simulink model "intercept_system"  (R2026b)
settings: Solver=ode4  StopTime=50  FixedStep=0.001
libraries: simulink x1
settings Model: Creator=rohan  LastModifiedBy=rohan

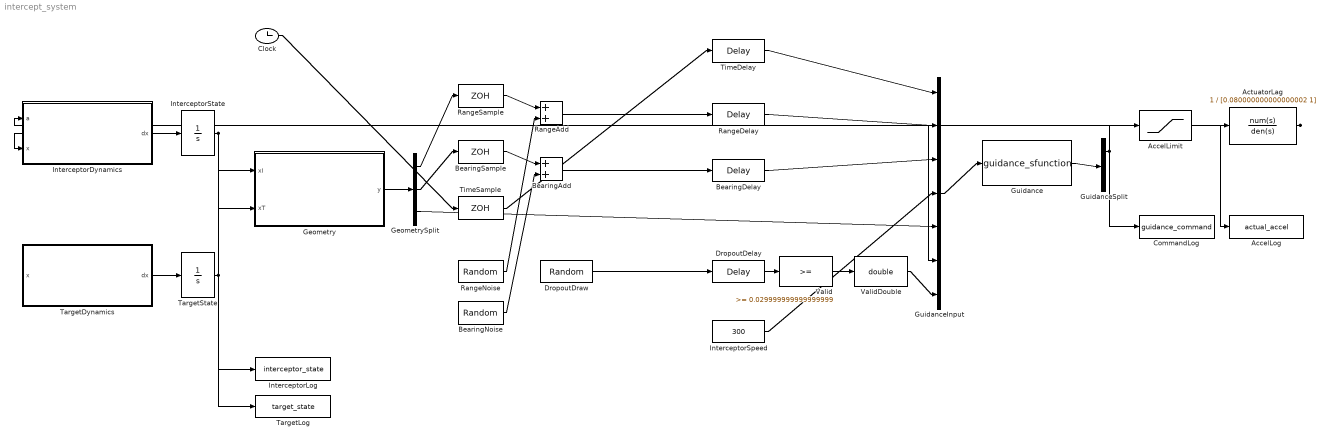
== system intercept_system ==
  AccelLimit : Saturate  UpperLimit=80  LowerLimit=-80
  AccelLog : ToWorkspace  VariableName=actual_accel  SaveFormat=Structure With Time  SampleTime=-1
  ActuatorLag : TransferFcn  Numerator=1  Denominator=[0.080000000000000002 1]
  BearingAdd : Sum
  BearingDelay : TransportDelay  DelayTime=0.080000000000000002
  BearingNoise : RandomNumber  Variance=1.5999999999999999e-05  Seed=565608883  SampleTime=0.02
  BearingSample : ZeroOrderHold  SampleTime=0.02
  Clock : Clock
  CommandLog : ToWorkspace  VariableName=guidance_command  SaveFormat=Structure With Time  SampleTime=-1
  DropoutDelay : TransportDelay  DelayTime=0.080000000000000002
  DropoutDraw : UniformRandomNumber  Minimum=0  Seed=2101286947  SampleTime=0.02
  Geometry : MATLAB Function  TreatAsAtomicUnit=on
  GeometrySplit : Demux  Outputs=3
  Guidance : S-Function  FunctionName=guidance_sfunction  Parameters='C:\Users\rohan\Downloads\seeker-intercept-guidance-complete\config\experiment.json'  SFunctionDeploymentMode=off  EnableBusSupport=off
  GuidanceInput : Mux  Inputs=7
  GuidanceSplit : Demux  Outputs=2
  InterceptorDynamics : MATLAB Function  TreatAsAtomicUnit=on
  InterceptorLog : ToWorkspace  VariableName=interceptor_state  SaveFormat=Structure With Time  SampleTime=-1
  InterceptorSpeed : Constant  Value=300
  InterceptorState : Integrator  InitialCondition=[0;0;0]
  RangeAdd : Sum
  RangeDelay : TransportDelay  DelayTime=0.080000000000000002
  RangeNoise : RandomNumber  Variance=25  Seed=2126880227  SampleTime=0.02
  RangeSample : ZeroOrderHold  SampleTime=0.02
  TargetDynamics : MATLAB Function  TreatAsAtomicUnit=on
  TargetLog : ToWorkspace  VariableName=target_state  SaveFormat=Structure With Time  SampleTime=-1
  TargetState : Integrator  InitialCondition=[4000;500;3.1415926535897931]
  TimeDelay : TransportDelay  DelayTime=0.080000000000000002
  TimeSample : ZeroOrderHold  SampleTime=0.02
  Valid : simulink/Logic and Bit Operations/Compare To Constant  relop=>=  const=0.029999999999999999  OutDataTypeStr=boolean
  ValidDouble : DataTypeConversion  OutDataTypeStr=double  SaturateOnIntegerOverflow=off  RndMeth=Floor
  wires:
  InterceptorDynamics/1(dx) -> InterceptorState/1
  InterceptorState/1 -> InterceptorDynamics/2(x), Geometry/1(xI), InterceptorLog/1
  TargetDynamics/1(dx) -> TargetState/1
  TargetState/1 -> TargetDynamics/1(x), Geometry/2(xT), TargetLog/1
  Geometry/1(y) -> GeometrySplit/1
  GeometrySplit/1 -> RangeSample/1
  GeometrySplit/2 -> BearingSample/1
  Clock/1 -> TimeSample/1
  RangeSample/1 -> RangeAdd/1
  RangeNoise/1 -> RangeAdd/2
  BearingSample/1 -> BearingAdd/1
  BearingNoise/1 -> BearingAdd/2
  TimeSample/1 -> TimeDelay/1
  RangeAdd/1 -> RangeDelay/1
  BearingAdd/1 -> BearingDelay/1
  DropoutDraw/1 -> DropoutDelay/1
  DropoutDelay/1 -> Valid/1
  Valid/1 -> ValidDouble/1
  TimeDelay/1 -> GuidanceInput/1
  RangeDelay/1 -> GuidanceInput/2
  BearingDelay/1 -> GuidanceInput/3
  InterceptorSpeed/1 -> GuidanceInput/4
  GeometrySplit/3 -> GuidanceInput/5
  GuidanceInput/1 -> Guidance/1
  Guidance/1 -> GuidanceSplit/1
  GuidanceSplit/1 -> AccelLimit/1, CommandLog/1
  AccelLimit/1 -> ActuatorLag/1
  ActuatorLag/1 -> InterceptorDynamics/1(a), GuidanceInput/6, AccelLog/1
  ValidDouble/1 -> GuidanceInput/7

== matlab function intercept_system/InterceptorDynamics ==
  data: a input; dx output; x input
function dx=f(a,x)
V=300; dx=[V*cos(x(3));V*sin(x(3));a/max(V,1e-9)];
end

== matlab function intercept_system/Geometry ==
  data: xI input; y output; xT input
function y=f(xI,xT)
r=xT(1:2)-xI(1:2); y=[hypot(r(1),r(2));atan2(r(2),r(1));xI(3)];
end

== matlab function intercept_system/TargetDynamics ==
  data: x input; dx output
function dx=f(x)
V=220; a=20; dx=[V*cos(x(3));V*sin(x(3));a/max(V,1e-9)];
end
